simulink library "pgctrl"  (R2016b)
settings: Solver=VariableStepAuto  StartTime=0.0  StopTime=10.0  RelTol=1e-3
values from neighbouring files (symbols this model uses):
  pglfd_damping_multiplier = 1.0    (= 1)    [init_pglfd.m]
undefined symbols (not defined in the file or in its folder): curl, DiscIntNeverNeededParam, manifold_stiffness_delay_buffer_size, R3, SO3
libraries: pgctrl x24, pgmanif x15, pgtrafo x10, simulink x8, simulink_need_slupdate x1
(part 2 of 2)

== system pgctrl/Precision to Stiffness/Delay Decrease ==
  kin : Inport
  delay : Inport  Port=2
  Delay : Delay  DelayLengthSource=Input port  DelayLengthUpperLimit=manifold_stiffness_delay_buffer_size  RemoveDelayLengthCheckInGeneratedCode=on  UseCircularBuffer=on
      settings: InputPortMap=u0,p1
  Delay k decrease : MATLAB Function  TreatAsAtomicUnit=on
  Saturation : Saturate  UpperLimit=manifold_stiffness_delay_buffer_size  LowerLimit=0
  Weighted Sample Time : SampleTimeMath  TsampMathOp=/  OutDataTypeStr=Inherit: Inherit via back propagation
  kdel : Outport
  del_out : Outport  Port=2
  wires:
  kin/1 -> Delay k decrease/1(kin), Delay/1
  delay/1 -> Weighted Sample Time/1
  Delay/1 -> Delay k decrease/2(kdel)
  Delay k decrease/1(kout) -> kdel/1
  Weighted Sample Time/1 -> Saturation/1
  Saturation/1 -> Delay k decrease/3(delay_steps), Delay/2
  Delay k decrease/2(delay_decrease) -> del_out/1

== system pgctrl/Precision to Stiffness/Dynamic Scaling ==
  k_scaled : Inport  Partition=on  PartitionDimension=1  PartitionWidth=1
  W : Inport  Port=2  Partition=on  PartitionDimension=2  PartitionWidth=1
  stiff_max : Inport  Port=3  Partition=on  PartitionDimension=1  PartitionWidth=1
  rot_max : Inport  Port=4  Partition=on  PartitionDimension=1  PartitionWidth=1
  kmin : Inport  Port=5
  For Each : ForEach  DisableCoverage=on  IndexMode=One-based
  Limit Rotational Stiffness : MATLAB Function  TreatAsAtomicUnit=on
  Saturation Dynamic1 : simulink/Discontinuities/Saturation Dynamic  OutMin=[]  OutMax=[]  OutDataTypeStr=Inherit: Same as second input  OutDataType=fixdt(1, 16)  OutScaling=2^-10  DoSatur=off
  k_sat : Outport  ConcatenationDimension=1
  wires:
  kmin/1 -> Saturation Dynamic1/3
  stiff_max/1 -> Limit Rotational Stiffness/2(stiff_max)
  rot_max/1 -> Limit Rotational Stiffness/3(rot_max)
  W/1 -> Limit Rotational Stiffness/1(W)
  Limit Rotational Stiffness/1(y) -> Saturation Dynamic1/1
  k_scaled/1 -> Saturation Dynamic1/2
  Saturation Dynamic1/1 -> k_sat/1

== system pgctrl/SE(3) Task Parameterization/SE(3) Rotation ==
  note: A Matrix: [R 0; 0 I]
  trafo : Inport
  Assignment : Assignment  NumberOfDimensions=2  DiagnosticForDimensions=Warning  IndexOptions=Index vector (dialog),Index vector (dialog)  Indices=1:3,1:3  OutputSizes=1,1
  Identity : Constant  Value=eye(6)
  extract quaternion : pgtrafo/extract quaternion
  quaternion to rotmat : pgtrafo/quaternion to rotmat
  rot : Outport
  wires:
  trafo/1 -> extract quaternion/1
  Identity/1 -> Assignment/1
  Assignment/1 -> rot/1
  quaternion to rotmat/1 -> Assignment/2
  extract quaternion/1 -> quaternion to rotmat/1

== system pgctrl/Manifold Impedance/Manifold Curl Stiffness/Enable ==
  singular : Inport
  Constant : Constant  Value=allow_asymmetric
  Logical Operator : Logic  Operator=OR  AllPortsSameDT=off  OutDataTypeStr=boolean
  Logical Operator1 : Logic  Operator=NOT  AllPortsSameDT=off  OutDataTypeStr=boolean
  enable : Outport
  wires:
  Logical Operator1/1 -> Logical Operator/2
  Constant/1 -> Logical Operator1/1
  singular/1 -> Logical Operator/1
  Logical Operator/1 -> enable/1

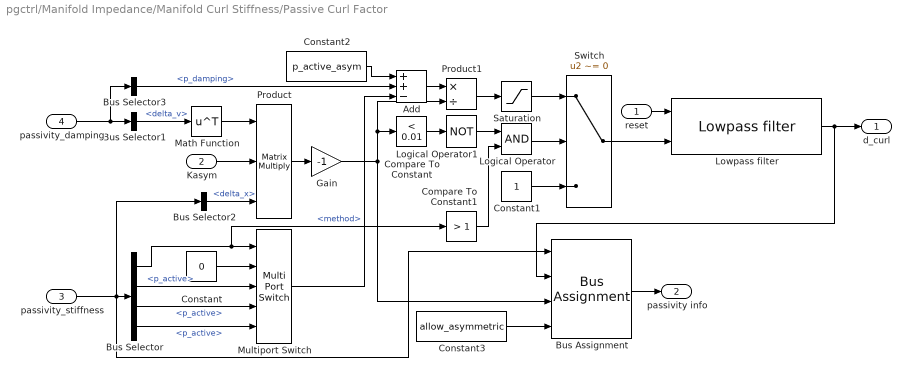
== system pgctrl/Manifold Impedance/Manifold Curl Stiffness/Passive Curl Factor ==
  reset : Inport
  Kasym : Inport  Port=2
  passivity_stiffness : Inport  Port=3
  passivity_damping : Inport  Port=4
  Add : Sum  Inputs=++-
  Bus Assignment : BusAssignment  AssignedSignals=curl.d,curl.p_active,curl.allow_asymmetric
  Bus Selector : BusSelector  OutputSignals=computed.method,k.p_active,l.p_active,l_disc.p_active
  Bus Selector1 : BusSelector  OutputSignals=delta_v
  Bus Selector2 : BusSelector  OutputSignals=computed.delta_x
  Bus Selector3 : BusSelector  OutputSignals=p_damping
  Compare To Constant : simulink/Logic and Bit Operations/Compare To Constant  relop=<  const=0.01  OutDataTypeStr=boolean
  Compare To Constant1 : simulink/Logic and Bit Operations/Compare To Constant  relop=>  const=1  OutDataTypeStr=boolean
  Constant : Constant  Value=0
  Constant1 : Constant
  Constant2 : Constant  Value=p_active_asym
  Constant3 : Constant  Value=allow_asymmetric  OutDataTypeStr=boolean
  Gain : Gain  Gain=-1
  Logical Operator : Logic  AllPortsSameDT=off  OutDataTypeStr=boolean
  Logical Operator1 : Logic  Operator=NOT  AllPortsSameDT=off  OutDataTypeStr=boolean
  Lowpass filter : pgtrafo/Lowpass filter  f_c=1
  Math Function : Math  Operator=transpose  SaturateOnIntegerOverflow=on
  Multiport Switch : MultiPortSwitch  Inputs=4
  Product : Product  Inputs=3  Multiplication=Matrix(*)
  Product1 : Product  Inputs=*/
  Saturation : Saturate  UpperLimit=1  LowerLimit=0
  Switch : Switch  Criteria=u2 ~= 0  Threshold=1
  d_curl : Outport  PortDimensions=1
  passivity info : Outport  Port=2  PortDimensions=1
  wires:
  Bus Selector/3 -> Multiport Switch/4  "<p_active>"
  Kasym/1 -> Product/2
  Product/1 -> Gain/1
  Bus Selector/1 -> Compare To Constant1/1, Multiport Switch/1  "<method>"
  Multiport Switch/1 -> Add/3
  Bus Selector/2 -> Multiport Switch/3  "<p_active>"
  Bus Selector3/1 -> Add/2  "<p_damping>"
  Bus Selector/4 -> Multiport Switch/5  "<p_active>"
  Bus Selector1/1 -> Math Function/1  "<delta_v>"
  Bus Selector2/1 -> Product/3  "<delta_x>"
  passivity_damping/1 -> Bus Selector3/1, Bus Selector1/1
  passivity_stiffness/1 -> Bus Selector2/1, Bus Assignment/1, Bus Selector/1
  Add/1 -> Product1/1
  Math Function/1 -> Product/1
  Constant/1 -> Multiport Switch/2
  Saturation/1 -> Switch/1
  Product1/1 -> Saturation/1
  Constant1/1 -> Switch/3
  Bus Assignment/1 -> passivity info/1
  Compare To Constant/1 -> Logical Operator1/1
  Logical Operator1/1 -> Logical Operator/1
  Logical Operator/1 -> Switch/2
  Lowpass filter/1 -> d_curl/1, Bus Assignment/2
  Compare To Constant1/1 -> Logical Operator/2
  Constant2/1 -> Add/1
  Gain/1 -> Compare To Constant/1, Product1/2, Bus Assignment/3
  Switch/1 -> Lowpass filter/2
  reset/1 -> Lowpass filter/1
  Constant3/1 -> Bus Assignment/4

== system pgctrl/Manifold Stiffness/Passivity Controller/Curl Empty Info ==
  Bus Creator3 : BusCreator  Inputs=3
  Constant : Constant  Value=0
  Constant4 : Constant  Value=0
  Constant8 : Constant  Value=0  OutDataTypeStr=boolean
  curl : Outport
  wires:
  Constant8/1 -> Bus Creator3/1  "allow_asymmetric"
  Bus Creator3/1 -> curl/1
  Constant/1 -> Bus Creator3/2  "p_active"
  Constant4/1 -> Bus Creator3/3  "d"

== system pgctrl/Manifold Stiffness/Passivity Controller/Damping Power Augmentation ==
  note: Limit power derivative
      | to initial_energy .
  reset : Inport
  P_damping : Inport  Port=2
  P_active : Inport  Port=3
  Add : Sum  Inputs=+-
  Add1 : Sum
  Constant : Constant  Value=initial_energy
  Discrete-Time Integrator : DiscreteIntegrator  ExternalReset=either  InitialConditionSource=external  InitialConditionSetting=State (most efficient)  SampleTime=-1  LimitOutput=on  UpperSaturationLimit=initial_energy  LowerSaturationLimit=0  ICPrevOutput=DiscIntNeverNeededParam  ICPrevScaledInput=DiscIntNeverNeededParam
  Saturation : Saturate  UpperLimit=0  LowerLimit=-inf
  Saturation1 : Saturate  UpperLimit=initial_power  LowerLimit=0
  Weighted Sample Time : SampleTimeMath  TsampMathOp=/
  P_avail : Outport
  initial_energy : Outport  Port=2
  wires:
  Constant/1 -> Discrete-Time Integrator/3
  reset/1 -> Discrete-Time Integrator/2
  P_damping/1 -> Add1/1, Add/1
  P_active/1 -> Add/2
  Add/1 -> Saturation/1
  Saturation/1 -> Discrete-Time Integrator/1
  Discrete-Time Integrator/1 -> initial_energy/1, Weighted Sample Time/1
  Weighted Sample Time/1 -> Saturation1/1
  Add1/1 -> P_avail/1
  Saturation1/1 -> Add1/2

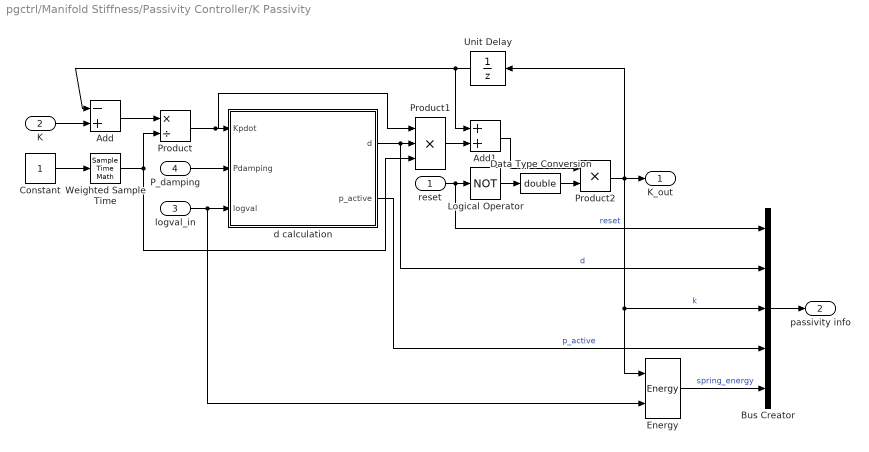
== system pgctrl/Manifold Stiffness/Passivity Controller/K Passivity ==
  reset : Inport
  K : Inport  Port=2
  logval_in : Inport  Port=3
  P_damping : Inport  Port=4
  Add : Sum  Inputs=-+
  Add1 : Sum
  Bus Creator : BusCreator  Inputs=5  OutDataTypeStr=Bus: bus_manifold_passivity_k
  Constant : Constant
  Data Type Conversion : DataTypeConversion  OutDataTypeStr=double
  Energy : pgctrl/Energy
  Logical Operator : Logic  Operator=NOT  AllPortsSameDT=off  OutDataTypeStr=boolean
  Product : Product  Inputs=*/
  Product1 : Product  Inputs=3
  Product2 : Product
  Unit Delay : UnitDelay  SampleTime=-1
  Weighted Sample Time : SampleTimeMath  TsampMathOp=Ts Only
  d calculation : MATLAB Function  TreatAsAtomicUnit=on
  K_out : Outport
  passivity info : Outport  Port=2  OutDataTypeStr=Bus: bus_manifold_passivity_k
  wires:
  Constant/1 -> Weighted Sample Time/1
  K/1 -> Add/2
  Unit Delay/1 -> Add1/1, Add/1
  Add/1 -> Product/1
  Weighted Sample Time/1 -> Product/2, Product1/3
  d calculation/1(d) -> Bus Creator/2, Product1/2  "d"
  Product/1 -> Product1/1, d calculation/1(Kpdot)
  Product1/1 -> Add1/2
  P_damping/1 -> d calculation/2(Pdamping)
  reset/1 -> Bus Creator/1, Logical Operator/1  "reset"
  Logical Operator/1 -> Data Type Conversion/1
  Data Type Conversion/1 -> Product2/2
  Add1/1 -> Product2/1
  Bus Creator/1 -> passivity info/1
  d calculation/2(p_active) -> Bus Creator/4  "p_active"
  Product2/1 -> Energy/1, Bus Creator/3, Unit Delay/1, K_out/1  "k"
  logval_in/1 -> Energy/2, d calculation/3(logval)
  Energy/1 -> Bus Creator/5  "spring_energy"

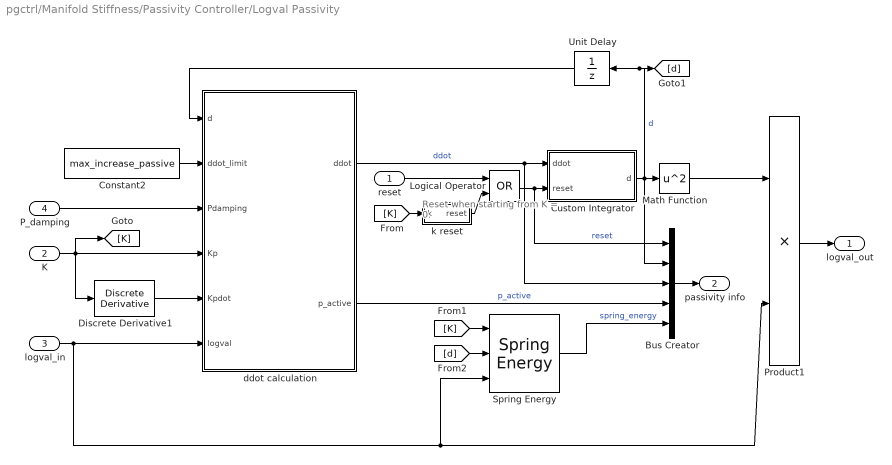
== system pgctrl/Manifold Stiffness/Passivity Controller/Logval Passivity ==
  note: Reset when starting from K = 0.
  reset : Inport
  K : Inport  Port=2
  logval_in : Inport  Port=3
  P_damping : Inport  Port=4
  Bus Creator : BusCreator  Inputs=5  OutDataTypeStr=Bus: bus_manifold_passivity_l
  Constant2 : Constant  Value=max_increase_passive
  Custom Integrator : Subsystem
  Discrete Derivative1 : simulink/Discrete/Discrete Derivative  gainval=1.0  ICPrevScaledInput=0.0  OutMin=[]  OutMax=[]  OutDataType=fixdt(1, 16)  OutScaling=2^-10  DoSatur=off
  Logical Operator : Logic  Operator=OR  AllPortsSameDT=off  OutDataTypeStr=boolean
  Math Function : Math  Operator=square  SaturateOnIntegerOverflow=on
  Product1 : Product
  Spring Energy : pgctrl/Spring Energy
  Unit Delay : UnitDelay  SampleTime=-1
  ddot calculation : MATLAB Function  TreatAsAtomicUnit=on
  k reset : Subsystem
  logval_out : Outport
  passivity info : Outport  Port=2  OutDataTypeStr=Bus: bus_manifold_passivity_l
  wires:
  logval_in/1 -> ddot calculation/6(logval), Spring Energy/3, Product1/2
  P_damping/1 -> ddot calculation/3(Pdamping)
  K/1 -> [K], Discrete Derivative1/1, ddot calculation/4(Kp)
  ddot calculation/1(ddot) -> Custom Integrator/1(ddot), Bus Creator/3  "ddot"
  Custom Integrator/1(d) -> Bus Creator/2, Unit Delay/1, [d], Math Function/1  "d"
  Discrete Derivative1/1 -> ddot calculation/5(Kpdot)
  Product1/1 -> logval_out/1
  Constant2/1 -> ddot calculation/2(ddot_limit)
  Math Function/1 -> Product1/1
  Logical Operator/1 -> Bus Creator/1, Custom Integrator/2(reset)  "reset"
  Unit Delay/1 -> ddot calculation/1(d)
  reset/1 -> Logical Operator/1
  [K] -> k reset/1(k)
  k reset/1(reset) -> Logical Operator/2
  Bus Creator/1 -> passivity info/1
  Spring Energy/1 -> Bus Creator/5  "spring_energy"
  ddot calculation/2(p_active) -> Bus Creator/4  "p_active"
  [K] -> Spring Energy/1
  [d] -> Spring Energy/2

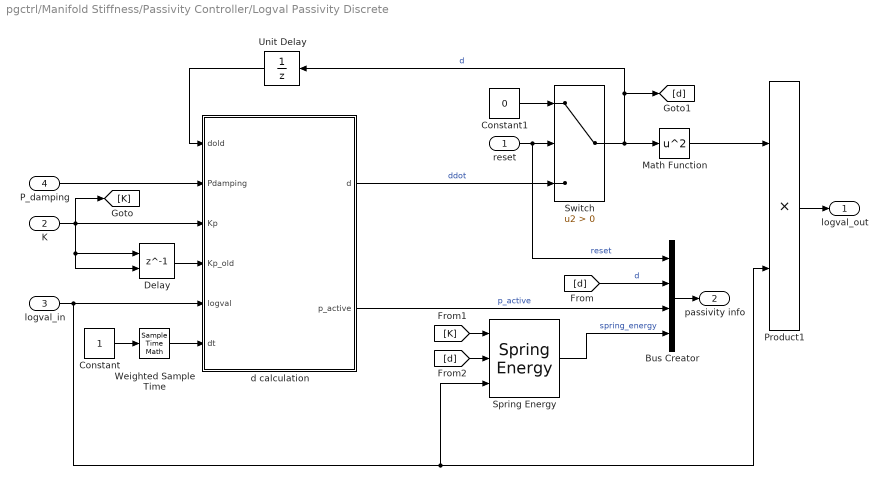
== system pgctrl/Manifold Stiffness/Passivity Controller/Logval Passivity Discrete ==
  reset : Inport
  K : Inport  Port=2
  logval_in : Inport  Port=3
  P_damping : Inport  Port=4
  Bus Creator : BusCreator  Inputs=4  OutDataTypeStr=Bus: bus_manifold_passivity_l_discrete
  Constant : Constant
  Constant1 : Constant  Value=0
  Delay : Delay  DelayLength=1  InitialConditionSource=Input port
      settings: InputPortMap=u0,p4
  Math Function : Math  Operator=square  SaturateOnIntegerOverflow=on
  Product1 : Product
  Spring Energy : pgctrl/Spring Energy
  Switch : Switch  Criteria=u2 > Threshold
  Unit Delay : UnitDelay  SampleTime=-1
  Weighted Sample Time : SampleTimeMath  TsampMathOp=Ts Only
  d calculation : MATLAB Function  TreatAsAtomicUnit=on
  logval_out : Outport
  passivity info : Outport  Port=2  OutDataTypeStr=Bus: bus_manifold_passivity_l_discrete
  wires:
  [d] -> Spring Energy/2
  [K] -> Spring Energy/1
  d calculation/2(p_active) -> Bus Creator/3  "p_active"
  Spring Energy/1 -> Bus Creator/4  "spring_energy"
  Bus Creator/1 -> passivity info/1
  reset/1 -> Bus Creator/1, Switch/2  "reset"
  Unit Delay/1 -> d calculation/1(dold)
  Math Function/1 -> Product1/1
  Product1/1 -> logval_out/1
  Switch/1 -> Math Function/1, [d], Unit Delay/1  "d"
  d calculation/1(d) -> Switch/3  "ddot"
  K/1 -> Delay/2, Delay/1, [K], d calculation/3(Kp)
  P_damping/1 -> d calculation/2(Pdamping)
  logval_in/1 -> Product1/2, Spring Energy/3, d calculation/5(logval)
  Weighted Sample Time/1 -> d calculation/6(dt)
  Constant/1 -> Weighted Sample Time/1
  Constant1/1 -> Switch/1
  [d] -> Bus Creator/2  "d"
  Delay/1 -> d calculation/4(Kp_old)

== system pgctrl/Manifold Stiffness/Passivity Controller/None Info ==
  k : Inport
  dx : Inport  Port=2
  Bus Creator : BusCreator  Inputs=2  OutDataTypeStr=Bus: bus_manifold_passivity_none
  Discrete Derivative : simulink/Discrete/Discrete Derivative  gainval=1.0  ICPrevScaledInput=0.0  OutMin=[]  OutMax=[]  OutDataType=fixdt(1, 16)  OutScaling=2^-10  DoSatur=off
  Energy : pgctrl/Energy
  Power : pgctrl/Energy
  none : Outport
  wires:
  k/1 -> Energy/1, Discrete Derivative/1
  dx/1 -> Power/2, Energy/2
  Bus Creator/1 -> none/1
  Energy/1 -> Bus Creator/2  "spring_energy"
  Power/1 -> Bus Creator/1  "p_active"
  Discrete Derivative/1 -> Power/1

== system pgctrl/Manifold Stiffness/Passivity Controller/Logval Passivity/Custom Integrator ==
  ddot : Inport
  reset : Inport  Port=2
  Add : Sum
  Constant : Constant
  Data Type Conversion : DataTypeConversion  OutDataTypeStr=double
  Logical Operator : Logic  Operator=NOT  AllPortsSameDT=off  OutDataTypeStr=boolean
  Product : Product
  Saturation : Saturate  UpperLimit=1  LowerLimit=0
  Switch : Switch  Criteria=u2 > Threshold
  Unit Delay Resettable External IC1 : simulink_need_slupdate/Unit Delay Resettable External IC  tsamp=-1
  Weighted Sample Time : SampleTimeMath  TsampMathOp=Ts Only
  d : Outport
  wires:
  Logical Operator/1 -> Data Type Conversion/1
  ddot/1 -> Product/1
  Data Type Conversion/1 -> Unit Delay Resettable External IC1/3, Switch/1
  reset/1 -> Logical Operator/1, Unit Delay Resettable External IC1/2, Switch/2
  Switch/1 -> Saturation/1
  Constant/1 -> Weighted Sample Time/1
  Weighted Sample Time/1 -> Product/2
  Product/1 -> Add/1
  Unit Delay Resettable External IC1/1 -> Add/2
  Add/1 -> Switch/3
  Saturation/1 -> Unit Delay Resettable External IC1/1, d/1

== system pgctrl/Manifold Stiffness/Passivity Controller/Logval Passivity/k reset ==
  k : Inport
  Abs : Abs
  Compare To Constant : simulink/Logic and Bit Operations/Compare To Constant  relop=<=  const=0.01  OutDataTypeStr=boolean
  Sum of Elements : Sum  Inputs=+
  reset : Outport
  wires:
  Compare To Constant/1 -> reset/1
  k/1 -> Abs/1
  Sum of Elements/1 -> Compare To Constant/1
  Abs/1 -> Sum of Elements/1

== matlab function pgctrl/Double Diagonalization Damping Design/Damping Design using Double Diagonalization/Damping Design ==
  data: K input; M input; D output; zeta input
function D = damping_design(K, M, zeta)

[Vmat, Dmat] = eig(K, M); % generalized eigenvalue problem
D = 2*zeta*M*real(Vmat)*real(sqrt(Dmat))/real(Vmat);
% Vmat = inv(Q'); M = Q*Q' -> Q = M*Vmat

%[Q, Dmat] = double_diagonalization(M, K);
%D = 2*zeta*Q*real(sqrt(Dmat))*Q';

== matlab function pgctrl/inv ==
  data: u input; y output
function y = inverse(u)

y = inv(u);

== matlab function pgctrl/Manifold Stiffness/Passivity Controller/Logval Passivity Discrete/d calculation ==
  data: dold input; Pdamping input; Kp input; Kp_old input; logval input; dt input; d output; p_active output
function [d, p_active] = passivize_limit_length_discrete(dold, Pdamping, Kp, Kp_old, logval, dt)

% calculate new d with new logval
d = min(max(sqrt((0.5*dold^2*logval'*Kp_old*logval + Pdamping*dt) / (0.5*logval'*Kp*logval + eps)), 0), 1);

% calculate active power from the change in Kp and d
p_active = (0.5*d^2*logval'*Kp*logval - 0.5*dold^2*logval'*Kp_old*logval) / dt;

== matlab function pgctrl/Precision to Stiffness/Delay Decrease/Delay k decrease ==
  data: kin input; kout output; kdel input; delay_steps input; delay_decrease output
 function [kout, delay_decrease] = delayed_k(kin, kdel, delay_steps)

%% persistent variables
persistent last_k;
if isempty(last_k)
    last_k = kin;
end

persistent first_decrease_k;
if isempty(first_decrease_k)
    first_decrease_k = kin;
end

persistent decrease_counter;
if isempty(decrease_counter)
    decrease_counter = zeros(size(kin));
end


%% check if decreasing
kout = kin; % pre-assign
delay_decrease = false;
for i=1:size(kin,1)
    if kin(i) < last_k(i)
        % save current k if first decrease
        if decrease_counter(i) == 0
            first_decrease_k(i) = last_k(i);
        end
        
        if decrease_counter(i) >= delay_steps
            % decrease with delay
            kout(i) = kdel(i);
        else
            % hold if delay too low
            kout(i) = first_decrease_k(i);
        end
        
        decrease_counter(i) =  decrease_counter(i) + 1;
        delay_decrease = true;
    else
        decrease_counter(i) = 0;
    end
end


%% assign state
last_k = kout;

== matlab function pgctrl/Stiffness Adaptation/Stiffness Adaptation ==
  data: Kin input; Kadap output; pose_in input; manifold_id parameter
function Kadap = stiffness_adaptation(Kin, pose_in, manifold_id)

% preset the output
Kadap = Kin;

% adapt to the radius
if manifold_id == 1
    r = pose_in(3);
    Kadap(1,1) = Kadap(1,1) * r^2;
elseif manifold_id == 2
    r = pose_in(4);
    Kadap(1,1) = Kadap(1,1) * r^2;
    Kadap(2,2) = Kadap(2,2) * r^2;
end

== matlab function pgctrl/Manifold Velocity Control/inv ==
  data: u input; y output
function y = inverse(u)

y = inv(u);

== matlab function pgctrl/Matrix Nonzero/Matrix Nonzero ==
  data: u input; y output
function y = fcn(u)
%#codegen

y = any(any(u));

== matlab function pgctrl/Precision to Stiffness/get diagonal ==
  data: u input; y output
function y = get_diag(u)

y = diag(u);

== matlab function pgctrl/Precision to Stiffness/stiffness max values ==
  data: K_diag input; kmax_trans output; R input; kmax_rot output
function [kmax_trans, kmax_rot] = stiffness_max_values(K_diag, R)

% first translations
% translations are a diag([x, y, z]) so we can limit individual dofs
kdiag_trans_rot = diag(R(1:3,1:3)'*diag(K_diag(1:3))*R(1:3,1:3));
kdiag_trans_rotback = diag(R(1:3,1:3)*diag(kdiag_trans_rot)*R(1:3,1:3)');
fac = min(max(kdiag_trans_rotback./K_diag(1:3)), 1);
kmax_trans = kdiag_trans_rot / fac;

% then rotations
% don't do anything here, rotations are not an id matrix
kmax_rot = K_diag(4:6);

%% old code
% first translations
%R_trans = R(1:3, 1:3);
%kmax_trans = sqrt(sum((R_trans * diag(K_diag(1:3))).^2, 1))';
%for i=1:3
%    kmax_trans = min(kmax_trans, (repmat(K_diag(i) + 1e-3, 1, 3) ./ abs(R_trans(i, :) + 1e-12))');
%end

% then rotations
%R_rot = R(4:6, 4:6);
%kmax_rot = sqrt(sum((R_rot * diag(K_diag(4:6))).^2, 1))';
%for i=1:3
%    kmax_rot = min(kmax_rot, (repmat(K_diag(i + 3) + 1e-3, 1, 3) ./ abs(R_rot(i, :) + 1e-12))');
%end

== matlab function pgctrl/Precision from R3*SO(3)/inverse ==
  data: singular input; u input; y output
function y = inv(singular, u)

if singular
    y = zeros(size(u));
else
    y = inv(u);
end

== matlab function pgctrl/Manifold Stiffness/Passivity Controller/Logval Passivity/ddot calculation ==
  data: d input; ddot_limit input; Pdamping input; Kp input; Kpdot input; ddot output; logval input; p_active output
function [ddot, p_active] = passivize_limit_length(d, ddot_limit, Pdamping, Kp, Kpdot, logval)

% original length of the difference
orig_len = sqrt(logval'*logval);

% modify length only if we have a spring elongation
if orig_len > 1e-6
    ddot = (Pdamping - 0.5*d^2*(logval'*Kpdot*logval)) / (d*(logval'*Kp*logval) + 1e-10);
else
    ddot = 0;
end

% ensure ddot is valid
ddot = min(ddot, ddot_limit);
if ~isfinite(ddot)
    ddot = 0;
end

% calculate active power
p_active = 0.5*d^2*(logval'*Kpdot*logval) + ddot*d*(logval'*Kp*logval);

== matlab function pgctrl/Manifold Stiffness/Passivity Controller/K Passivity/d calculation ==
  data: Kpdot input; Pdamping input; d output; logval input; p_active output
function [d, p_active] = k_passivity(Kpdot, Pdamping, logval)

% calculate p_active from Kpdot
p_active = 0.5*logval'*Kpdot*logval;

if p_active > 0
    d = min(Pdamping / p_active, 1);
else
    d = 1;
end

% modulate p_active with d
p_active = d * p_active;

== matlab function pgctrl/Resymmetrize Matrix ==
  data: mat input; mat_repair output; is_symmetric output; zero_thresh input
function [mat_repair, is_symmetric] = repair(mat, zero_thresh)

is_symmetric = all(all(mat - mat' < 1e-5));

mat_repair = 0.5 * (mat + mat');
mat_repair(abs(mat_repair) < zero_thresh) = 0;

== matlab function pgctrl/Precision to Stiffness/Decompose P ==
  data: P input; Ps output; Pt output
function [Ps, Pt] = decompose_p(P)

P = 0.5 * (P + P');
Ps = P;
Pt = zeros(6,6);

Ps(4:6, 4:6) = Ps(4:6, 1:3) / Ps(1:3, 1:3) * Ps(1:3, 4:6);
Ps(~isfinite(Ps)) = 0;
Pt(4:6, 4:6) = P(4:6, 4:6) - Ps(4:6, 4:6);

Ps(abs(Ps) < 1e-3) = 0;
Pt(abs(Pt) < 1e-3) = 0;

== matlab function pgctrl/Precision to Stiffness/Decompose Ps ==
  data: k output; Ps input; W output
function [k, W] = decompose_ps(Ps)

k = diag(Ps(1:3, 1:3));

W = zeros(6, 3);
W(1:3, 1) = [1 0 0];
W(1:3, 2) = [0 1 0];
W(1:3, 3) = [0 0 1];

W(4:6, :) = Ps(4:6, 1:3) * diag(k.^-1);
W(~isfinite(W)) = 0;

== matlab function pgctrl/Precision to Stiffness/P_trans to R ==
  data: P_trans input; R output
function R = get_rotmat(P_trans)

[V, ~] = eig(P_trans);
R = blkdiag(real(V), real(V));

== matlab function pgctrl/Precision to Stiffness/Decompose Pt ==
  data: Pt input; k output; W output
function [k, W] = decompose_pt(Pt)

[V, D] = eig(Pt(4:6, 4:6));

k = diag(real(D));
W = zeros(6, 3);
W(4:6, :) = real(V);

== matlab function pgctrl/Precision to Stiffness/Create Stiffness ==
  data: k input; K output; W input
function K = create_k(k, W)

K = zeros(6, 6);
for i=1:6
    K = K + k(i) * W(:, i) * W(:, i)';
end

== matlab function pgctrl/Precision to Stiffness/Ensure Finite ==
  data: u input; y output
function y = ensure_finite(u)

y = u;
y(~isfinite(u)) = 0;

== matlab function pgctrl/Precision to Stiffness/Dynamic Scaling/Limit Rotational Stiffness ==
  data: y output; W input; stiff_max input; rot_max input
function y = limit_rot_stiffness(W, stiff_max, rot_max)

len_rot = W(4:6)'*W(4:6);
y = min(stiff_max, rot_max / len_rot);
